simulink library "lib_IC_VSM"  (R2026a)
settings: Solver=VariableStepAuto
undefined symbols (not defined in the file): block_buses, block_DC_buses, block_DC_toM, block_idx, block_toM, buses_lf, DC, dparams, fb, fref, iC, inv2Hv, invL, iR, iTf, omegab, op_intconv_VSM
libraries: sl_discontinuities x1
(part 3 of 3)

== system lib_IC_VSM/intconv_VSM/VCC/dynamic_limiting/VI/WOF_q/Bypass ==
  In1 : Inport
  Out1 : Outport
  wires:
  In1/1 -> Out1/1

== system lib_IC_VSM/intconv_VSM/VCC/dynamic_limiting_P/VI/WOF_d/Active ==
  In1 : Inport
  Impl : Subsystem
  Out1 : Outport
  wires:
  Impl/1(Out1) -> Out1/1
  In1/1 -> Impl/1(In1)

== system lib_IC_VSM/intconv_VSM/VCC/dynamic_limiting_P/VI/WOF_d/Bypass ==
  In1 : Inport
  Out1 : Outport
  wires:
  In1/1 -> Out1/1

== system lib_IC_VSM/intconv_VSM/VCC/dynamic_limiting_P/VI/WOF_q/Active ==
  In1 : Inport
  Impl : Subsystem
  Out1 : Outport
  wires:
  Impl/1(Out1) -> Out1/1
  In1/1 -> Impl/1(In1)

== system lib_IC_VSM/intconv_VSM/VCC/dynamic_limiting_P/VI/WOF_q/Bypass ==
  In1 : Inport
  Out1 : Outport
  wires:
  In1/1 -> Out1/1

== system lib_IC_VSM/intconv_VSM/VCC/dynamic_limiting/VI/WOF_d/Active/Impl ==
  In1 : Inport
  Gain : Gain  Gain=iTf
  I : Integrator  InitialConditionSource=external  InitialCondition=op_intconv_VSM.VCC_dynamic_limiting_VI_WOF_d_Active_Impl_I
  Sum : Sum  Inputs=+-|
  Sum4 : Sum  Inputs=|+-
  Out1 : Outport
  wires:
  Gain/1 -> I/1
  Sum4/1 -> Gain/1
  In1/1 -> I/2, Sum/1, Sum4/1
  I/1 -> Sum/2, Sum4/2
  Sum/1 -> Out1/1

== system lib_IC_VSM/intconv_VSM/VCC/dynamic_limiting/VI/WOF_q/Active/Impl ==
  In1 : Inport
  Gain : Gain  Gain=iTf
  I : Integrator  InitialConditionSource=external  InitialCondition=op_intconv_VSM.VCC_dynamic_limiting_VI_WOF_q_Active_Impl_I
  Sum : Sum  Inputs=+-|
  Sum4 : Sum  Inputs=|+-
  Out1 : Outport
  wires:
  Gain/1 -> I/1
  Sum4/1 -> Gain/1
  In1/1 -> I/2, Sum/1, Sum4/1
  I/1 -> Sum/2, Sum4/2
  Sum/1 -> Out1/1

== system lib_IC_VSM/intconv_VSM/VCC/dynamic_limiting_P/VI/WOF_d/Active/Impl ==
  In1 : Inport
  Gain : Gain  Gain=iTf
  I : Integrator  InitialConditionSource=external  InitialCondition=op_intconv_VSM.VCC_dynamic_limiting_P_VI_WOF_d_Active_Impl_I
  Sum : Sum  Inputs=+-|
  Sum4 : Sum  Inputs=|+-
  Out1 : Outport
  wires:
  Gain/1 -> I/1
  Sum4/1 -> Gain/1
  In1/1 -> I/2, Sum/1, Sum4/1
  I/1 -> Sum/2, Sum4/2
  Sum/1 -> Out1/1

== system lib_IC_VSM/intconv_VSM/VCC/dynamic_limiting_P/VI/WOF_q/Active/Impl ==
  In1 : Inport
  Gain : Gain  Gain=iTf
  I : Integrator  InitialConditionSource=external  InitialCondition=op_intconv_VSM.VCC_dynamic_limiting_P_VI_WOF_q_Active_Impl_I
  Sum : Sum  Inputs=+-|
  Sum4 : Sum  Inputs=|+-
  Out1 : Outport
  wires:
  Gain/1 -> I/1
  Sum4/1 -> Gain/1
  In1/1 -> I/2, Sum/1, Sum4/1
  I/1 -> Sum/2, Sum4/2
  Sum/1 -> Out1/1
